simulink model "RealTimeTarget"  (Simulink 7.5)
settings: Solver=FixedStepDiscrete  StartTime=0.0  StopTime=10.0  RelTol=1e-3
libraries: rtwinlib x2, simulink x1
settings Model: Creator=oded  LastModifiedBy=oded  SimulationMode=external
settings HardwareCC: ProdIntDivRoundTo=Zero  ProdEndianess=LittleEndian  ProdHWDeviceType=Generic->32-bit x86 compatible
settings RTWCC: SystemTargetFile=rtwin.tlc  TemplateMakefile=rtwin.tmf  Description=Real-Time Windows Target  ProcessScript=rtwin_make_rtw_hook  RTWCompilerOptimization=On
settings CodeAppCC: MaxIdLength=95
settings RTWinTargetCC: TargetFunctionLibrary=ANSI_C  ERTCodeCoverageTool=None  PortableWordSizes=off

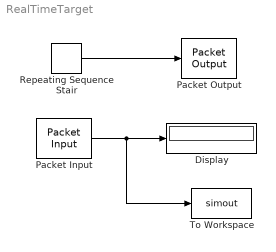
== system RealTimeTarget ==
  Display : Display
  Packet Input : rtwinlib/Packet Input  SampleTime=1  DrvAddress=0  DrvOptions=0  PacketSize=32  DataTypes='4*double'  ShowReady=off  ShowError=off  PacketID=1  ShowTimestamp=off
  Packet Output : rtwinlib/Packet Output  SampleTime=1  DrvAddress=0  DrvOptions=0  PacketSize=1  DataTypes='uint8'  ShowReady=off  ShowError=off  PacketID=1  InitialValue=[]  FinalValue=[]
  Repeating Sequence Stair : simulink/Sources/Repeating Sequence Stair  SystemSampleTime=-1  OutValues=[0 1 0 2 0 3 0 4 0 5 0 6].'  tsamp=-1  OutMin=[]  OutMax=[]  OutDataTypeStr=uint8  OutputDataTypeScalingMode=uint8  OutDataType=fixdt(0,8)  ConRadixGroup=Best Precision: Vector-wise  OutScaling=2^-12
  To Workspace : ToWorkspace  VariableName=simout  SampleTime=-1  SaveFormat=Structure
  wires:
  Repeating Sequence Stair/1 -> Packet Output/1
  Packet Input/1 -> Display/1, To Workspace/1
